simulink model "EINT_RL_closed_loop"  (R2025b)
settings: Solver=FixedStepAuto  StartTime=0.0  StopTime=T_end  FixedStep=Ts  RelTol=1e-3
values from neighbouring files (symbols this model uses):
  Ts = 0.05    [EINT_RL_eval.m]    (also in rl_controller.m)
settings Model: Creator=etienne  LastModifiedBy=etienne

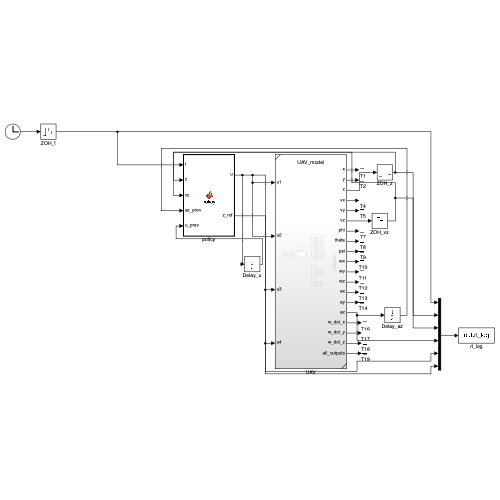
[thumbnail: Simulink's stored preview of the top-level diagram]
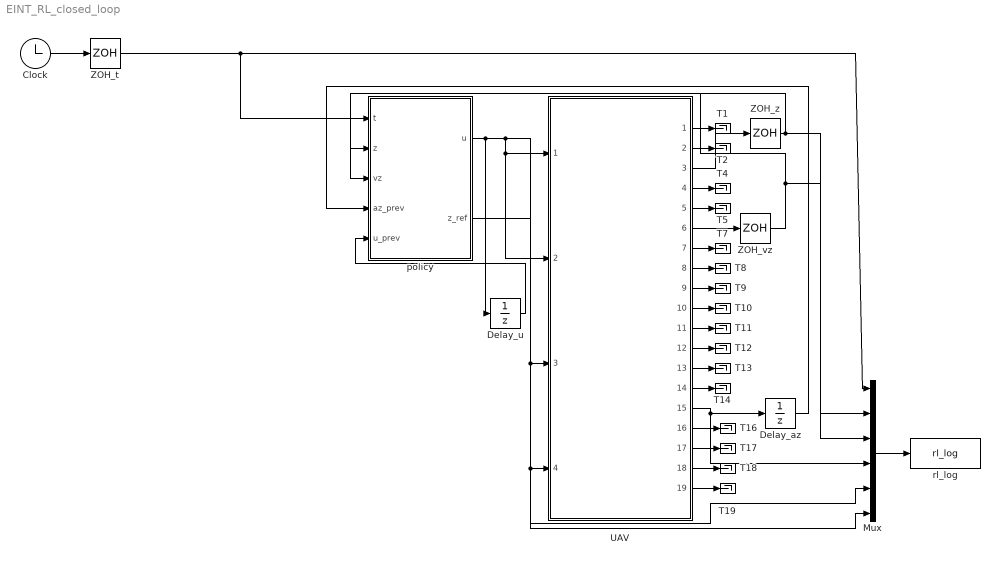
== system EINT_RL_closed_loop ==
  Clock : Clock
  Delay_az : UnitDelay  SampleTime=Ts  HasFrameUpgradeWarning=on
  Delay_u : UnitDelay  SampleTime=Ts  HasFrameUpgradeWarning=on
  Mux : Mux  Inputs=6
  T{1..2,4..5,7..14,16..19} (16 alike) : Terminator
  UAV : Subsystem  ReferencedSubsystem=UAV_model
  ZOH_t : ZeroOrderHold  SampleTime=Ts
  ZOH_vz : ZeroOrderHold  SampleTime=Ts
  ZOH_z : ZeroOrderHold  SampleTime=Ts
  policy : MATLAB Function  TreatAsAtomicUnit=on
  rl_log : ToWorkspace  VariableName=rl_log  SampleTime=Ts
  wires:
  Clock/1 -> ZOH_t/1
  UAV/3 -> ZOH_z/1
  UAV/6 -> ZOH_vz/1
  UAV/15 -> Mux/4, Delay_az/1
  ZOH_t/1 -> policy/1(t), Mux/1
  ZOH_z/1 -> policy/2(z), Mux/2
  ZOH_vz/1 -> policy/3(vz), Mux/3
  Delay_az/1 -> policy/4(az_prev)
  Delay_u/1 -> policy/5(u_prev)
  policy/1(u) -> UAV/1, UAV/2, UAV/4, Mux/5, UAV/3, Delay_u/1
  UAV/1 -> T1/1
  UAV/2 -> T2/1
  UAV/4 -> T4/1
  UAV/5 -> T5/1
  UAV/7 -> T7/1
  UAV/8 -> T8/1
  UAV/9 -> T9/1
  UAV/10 -> T10/1
  UAV/11 -> T11/1
  UAV/12 -> T12/1
  UAV/13 -> T13/1
  UAV/14 -> T14/1
  UAV/16 -> T16/1
  UAV/17 -> T17/1
  UAV/18 -> T18/1
  UAV/19 -> T19/1
  policy/2(z_ref) -> Mux/6
  Mux/1 -> rl_log/1

== matlab function EINT_RL_closed_loop/policy ==
  data: t input; u output; z input; vz input; az_prev input; u_prev input; z_ref output
function [u, z_ref] = policy(t, z, vz, az_prev, u_prev)
coder.extrinsic('rl_controller');
u = 0;
z_ref = 0;
[u, z_ref] = rl_controller(t, z, vz, az_prev, u_prev);
